simulink model "FullFMS_SIM_V0_1_5_R2025b"  (R2025b)
settings: Solver=FixedStepAuto  StopTime=inf  FixedStep=0.01  MaxStep=0.01  RelTol=1e-2
PreLoadFcn:
  | load("BUS_CONFIG_SIM.mat"); run("Param_SIM_V0_1_5.m")
libraries: opcualib x8
(part 2 of 2)

== stateflow chart FullFMS_SIM_V0_1_5_R2025b/Chart_SIM ==
  settings: updateMethod=DISCRETE  sampleTime=Ts_SIM
  state Conveyor29 [parallel]
    settings: executionOrder=1
    state Idle
      entry: SimSensors_20.SS_29_Cart_Stat=false; SimSensors_20.SS_29_Optic=false; SimSensors_20.SS_29_Cart_Next=false;
    state Arriving
      entry: SimSensors_20.SS_29_Cart_Next=true; SimActuators_20.SA_20_Conveyor=true; SimSensors_20.SS_20_Controler_On=true;
    state AtStop
      entry: SimSensors_20.SS_29_Cart_Next=false; SimSensors_20.SS_29_Count=true; SimSensors_20.SS_29_Cart_Stat=true; SimSensors_20.SS_29_Optic=true;
      PartOnCart=true; CartAt29=true; SimActuators_20.SA_20_Conveyor=false;
    state Delivered
      entry: SimSensors_20.SS_29_Count=false; SimControl_20.SC_29_CartDel=true; CRouteIn54=true; SimASi_50.SR_54_CRoute_In=true;
      during: SimSensors_20.SS_29_Optic = PartOnCart;
    state Leaving
      entry: SimControl_20.SC_29_CartDel=false; CRouteIn54=false; SimASi_50.SR_54_CRoute_In=false; CartAt29=false;
    (default) -> Idle
    Leaving -> Idle : after(t_leave,sec)
    Idle -> Arriving : [nCart < N_PARTS]
    Arriving -> AtStop : after(t_conv,sec)
    AtStop -> Delivered : after(T_CONV_T6,sec)
    Delivered -> Leaving : [SimASi_50.SR_54_CRoute_Out]
  state HD1_Ctrl [parallel]
    settings: executionOrder=2
    state Init
      entry: SimControl_50.SC_52_Profibus=true; SimControl_50.SC_55_PD_Sort=false; SimASi_50.SR_54_CRoute_Out=false;
      SimActuators_50.SA_50_Claw_Down=false; SimActuators_50.SA_50_Close_Claw=false; SimActuators_50.SA_50_Claw_2_Del=false; SimActuators_50.SA_50_Claw_2_Cart=false;
    state Ready
      entry: SimControl_50.SC_55_Initialization=true;
    state N1_StartMove
      entry: SimControl_50.SC_55_PD_Sort=false;
    state N2_LowerClaw
      entry: SimActuators_50.SA_50_Claw_Down=true;
    state N3_CloseClaw
      entry: SimActuators_50.SA_50_Close_Claw=true;
    state N3_Raise
      entry: SimActuators_50.SA_50_Claw_Down=false;
    state N4_Claw2Del
      entry: SimActuators_50.SA_50_Claw_2_Cart=false; SimActuators_50.SA_50_Claw_2_Del=true;
    state N5_LowerClaw2
      entry: SimActuators_50.SA_50_Claw_Down=true;
    state N6_Release
      entry: SimActuators_50.SA_50_Close_Claw=false;
    state N6_Raise
      entry: SimActuators_50.SA_50_Claw_Down=false;
    state N7_PDSort
      entry: SimControl_50.SC_55_PD_Sort=true;
    state N8_Claw2Cart
      entry: SimActuators_50.SA_50_Claw_2_Del=false; SimActuators_50.SA_50_Claw_2_Cart=true; Claw2CartCmd=true;
    state N9_CRouteOut
      entry: SimActuators_50.SA_50_Claw_2_Cart=false; Claw2CartCmd=false; SimASi_50.SR_54_CRoute_Out=true;
      exit: SimASi_50.SR_54_CRoute_Out=false; nCart = nCart + 1;
    (default) -> Init
    Init -> Ready : [SimSensors_50.SS_50_Claw_Cart && SimSensors_50.SS_50_Claw_High && ~SimSensors_50.SS_50_Part_in_Claw]
    N9_CRouteOut -> Ready : after(T_HD1_T1,sec)
    Ready -> N1_StartMove : [CRouteIn54 && CartAt29 && SimSensors_20.SS_29_Optic && ~SimSensors_60.SS_60_SPart]
    N1_StartMove -> N2_LowerClaw : [~SimControl_50.SC_55_PD_Sort && SimSensors_50.SS_50_Claw_Cart && SimSensors_50.SS_50_Claw_High && ~SimSensors_50.SS_50_Part_in_Claw]
    N2_LowerClaw -> N3_CloseClaw : [SimSensors_50.SS_50_Claw_Cart && SimSensors_50.SS_50_Claw_Low]
    N3_CloseClaw -> N3_Raise : [SimSensors_50.SS_50_Part_in_Claw]
    N3_Raise -> N4_Claw2Del : [SimSensors_50.SS_50_Claw_High && SimSensors_50.SS_50_Part_in_Claw && ~SimSensors_50.SS_50_Claw_Del]
    N4_Claw2Del -> N5_LowerClaw2 : [SimSensors_50.SS_50_Claw_Del && SimSensors_50.SS_50_Claw_High && SimSensors_50.SS_50_Part_in_Claw]
    N5_LowerClaw2 -> N6_Release : [SimSensors_50.SS_50_Claw_Del && SimSensors_50.SS_50_Claw_Low]
    N6_Release -> N6_Raise : [~SimSensors_50.SS_50_Part_in_Claw]
    N6_Raise -> N7_PDSort : [SimSensors_50.SS_50_Claw_Del && SimSensors_50.SS_50_Claw_High && ~SimSensors_50.SS_50_Part_in_Claw]
    N7_PDSort -> N8_Claw2Cart
    N8_Claw2Cart -> N9_CRouteOut : [SimSensors_50.SS_50_Claw_Cart]
  state HD1_Plant [parallel]
    settings: executionOrder=3
    state Vertical [parallel]
      settings: executionOrder=1
      state High
        entry: SimSensors_50.SS_50_Claw_High=true; SimSensors_50.SS_50_Claw_Low=false;
      state GoingDown
        entry: SimSensors_50.SS_50_Claw_High=false;
      state Low
        entry: SimSensors_50.SS_50_Claw_Low=true;
      state GoingUp
        entry: SimSensors_50.SS_50_Claw_Low=false;
      (default) -> High
      GoingUp -> High [order 1] : after(t_v_up,sec)
      High -> GoingDown : [SimActuators_50.SA_50_Claw_Down]
      GoingUp -> GoingDown [order 2] : [SimActuators_50.SA_50_Claw_Down]
      GoingDown -> Low [order 1] : after(t_v_down,sec)
      GoingDown -> GoingUp [order 2] : [~SimActuators_50.SA_50_Claw_Down]
      Low -> GoingUp : [~SimActuators_50.SA_50_Claw_Down]
    state Horizontal [parallel]
      settings: executionOrder=2
      state AtCart
        entry: SimSensors_50.SS_50_Claw_Cart=true; SimSensors_50.SS_50_Claw_Del=false;
      state ToDel
        entry: SimSensors_50.SS_50_Claw_Cart=false;
      state AtDel
        entry: SimSensors_50.SS_50_Claw_Del=true;
      state ToCart
        entry: SimSensors_50.SS_50_Claw_Del=false;
      (default) -> AtCart
      ToCart -> AtCart : after(t_h_cart,sec)
      AtCart -> ToDel : [SimActuators_50.SA_50_Claw_2_Del]
      ToDel -> AtDel : after(t_h_del,sec)
      AtDel -> ToCart : [SimActuators_50.SA_50_Claw_2_Cart]
    state Gripper [parallel]
      settings: executionOrder=3
      state Empty
        entry: SimSensors_50.SS_50_Part_in_Claw=false;
      state Gripping
      state Holding
        entry: SimSensors_50.SS_50_Part_in_Claw=true; PartOnCart=false;
      state Releasing
      (default) -> HD1_Plant.Gripper.Empty
      Releasing -> HD1_Plant.Gripper.Empty : after(t_grip,sec){SimSensors_60.SS_60_SPart = SimSensors_60.SS_60_SPart || SimSensors_50.SS_50_Claw_Del;}
      HD1_Plant.Gripper.Empty -> Gripping : [SimActuators_50.SA_50_Close_Claw && SimSensors_50.SS_50_Claw_Low && SimSensors_50.SS_50_Claw_Cart && PartOnCart]
      Gripping -> Holding : after(t_grip,sec)
      Holding -> Releasing : [~SimActuators_50.SA_50_Close_Claw && SimSensors_50.SS_50_Claw_Low]
  state SORT_Ctrl [parallel]
    entry: SimControl_60.SC_62_Profibus=false; SimControl_60.SC_65_Initialization=false; SimControl_60.SC_65_ID_1=false; SimControl_60.SC_65_ID_2=false; SimControl_60.SC_65_Part_Sorted=false;
    SimControl_60.SC_65_RBS_Output = (SORT_MODE == 1); SimControl_60.SC_65_RSB_Output = (SORT_MODE == 2); SimControl_60.SC_65_BRS_Output = (SORT_MODE == 3); SimControl_60.SC_65_BSR_Output = (SORT_MODE == 4); SimControl_60.SC_65_SRB_Output = (SORT_MODE == 5); SimControl_60.SC_65_SBR_Output = (SORT_MODE == 6);
    SimActuators_60.SA_60_Conveyor=false; SimActuators_60.SA_60_P1=false; SimActuators_60.SA_60_P2=false; SimActuators_60.SA_60_Identify=false; SimActuators_60.SA_61_Led_Start=false; SimActuators_60.SA_61_Led_Reset=false; SimActuators_60.SA_61_Led_Extra1=false; SimActuators_60.SA_61_Led_Extra2=false; SimActuators_60.SA_61_Panel_O4=false; SimActuators_60.SA_61_Panel_O5=false; SimActuators_60.SA_61_Panel_O6=false; SimActuators_60.SA_61_Panel_O7=false;
    FBSel = (SORT_MODE == 1 && SimControl_60.SC_65_RBS_Output) || (SORT_MODE == 2 && SimControl_60.SC_65_RSB_Output) || (SORT_MODE == 3 && SimControl_60.SC_65_BRS_Output) || (SORT_MODE == 4 && SimControl_60.SC_65_BSR_Output) || (SORT_MODE == 5 && SimControl_60.SC_65_SRB_Output) || (SORT_MODE == 6 && SimControl_60.SC_65_SBR_Output);
    settings: executionOrder=4
    state FB1_Init [parallel]
      settings: executionOrder=1
      state FB1_N2_Check
        entry: SimControl_60.SC_62_Profibus=true; FB1Init=false; SimControl_60.SC_65_Initialization=false;
      state FB1_N3_ClearPart
        entry: FB1Conv=true; FB1IDPin=true;
      state FB1_N1_InitOk
        entry: FB1Init=true; SimControl_60.SC_65_Initialization=true;
      (default) -> SORT_Ctrl.FB1_Init.FB1_N2_Check
      FB1_N3_ClearPart -> SORT_Ctrl.FB1_Init.FB1_N2_Check : [FB1Conv && SimSensors_60.SS_60_Part_Pass]{FB1Conv=false; FB1IDPin=false;}
      FB1_N1_InitOk -> SORT_Ctrl.FB1_Init.FB1_N2_Check : [SimSensors_60.SS_61_Reset]{FB1Conv=false; FB1IDPin=false; TrigConv=false; Lever1=false; Lever2=false; PinSort=false; PartDel=false;}
      SORT_Ctrl.FB1_Init.FB1_N2_Check -> FB1_N1_InitOk [order 1] : [SimControl_60.SC_62_Profibus && ~FB1Conv && ~SimSensors_60.SS_60_SPart && ~SimSensors_60.SS_60_SInd && ~SimSensors_60.SS_60_SPhoto && ~SimSensors_60.SS_60_Part_Pass]
      SORT_Ctrl.FB1_Init.FB1_N2_Check -> FB1_N3_ClearPart [order 2] : [SimSensors_60.SS_60_SPart || SimSensors_60.SS_60_SInd || SimSensors_60.SS_60_SPhoto]
    state FB4_9_Sort [parallel]
      settings: executionOrder=2
      state OB1_N4_9_Select
      state N1_StartConv
        entry: TrigConv=true; SimControl_60.SC_65_ID_1=false; SimControl_60.SC_65_ID_2=false;
      state N2_Identify
        en, du: if SimSensors_60.SS_60_SInd, SimControl_60.SC_65_ID_1=false; SimControl_60.SC_65_ID_2=true;
        elseif SimSensors_60.SS_60_SPhoto, SimControl_60.SC_65_ID_1=true; SimControl_60.SC_65_ID_2=true;
        else, SimControl_60.SC_65_ID_1=true; SimControl_60.SC_65_ID_2=false; end
      state N3_SelectLever
        entry: cID = 0;
        if SimControl_60.SC_65_ID_1 && SimControl_60.SC_65_ID_2, cID = 1; elseif SimControl_60.SC_65_ID_1, cID = 2; elseif SimControl_60.SC_65_ID_2, cID = 3; end
        Lever1 = (cID == SORT_MAP(SORT_MODE,1)); Lever2 = (cID == SORT_MAP(SORT_MODE,2)); PassStr = (cID == SORT_MAP(SORT_MODE,3));
        during: if (Lever1 && SimSensors_60.SS_60_SL1_Fwd) || (Lever2 && SimSensors_60.SS_60_SL2_Fwd) || (PassStr && SimSensors_60.SS_60_SL1_Bck && SimSensors_60.SS_60_SL2_Bck), PinSort = true; end
      state N4_PartDel
        entry: PartDel=true; Lever1=false;
        if SORT_MODE ~= 3, Lever2=false; end
      state N5_ResetNext
        entry: TrigConv=false; PinSort=false; PartDel=false; Lever1=false; Lever2=false; PassStr=false;
      (default) -> OB1_N4_9_Select
      N5_ResetNext -> OB1_N4_9_Select
      OB1_N4_9_Select -> N1_StartConv : [FB1Init && FBSel && SimControl_50.SC_55_PD_Sort && SimSensors_50.SS_50_Claw_Del]
      N1_StartConv -> N2_Identify
      N2_Identify -> N3_SelectLever : after(T_SORT_ID - Ts_SIM,sec)
      N3_SelectLever -> N4_PartDel : [SimSensors_60.SS_60_Part_Pass]
      N4_PartDel -> N5_ResetNext
    state OB1_N10_11 [parallel]
      settings: executionOrder=3
      state N10_Wait
        entry: SimControl_60.SC_65_Part_Sorted=false;
      state N10_PartPass
      state N11_PartSorted
        entry: SimControl_60.SC_65_Part_Sorted=true;
      (default) -> N10_Wait
      N11_PartSorted -> N10_Wait : after(T_SORT_T7,sec)
      N10_Wait -> N10_PartPass : [SimSensors_60.SS_60_Part_Pass]
      N10_PartPass -> N11_PartSorted : [~SimSensors_60.SS_60_Part_Pass]
    state FB3_Actuators [parallel]
      settings: executionOrder=4
      state FB3_Map
        during: ConvOn60 = SimSensors_60.SS_61_Key_Pos && (TrigConv || FB1Conv); SimActuators_60.SA_60_Conveyor = ConvOn60;
        SimActuators_60.SA_60_P1 = SimSensors_60.SS_61_Key_Pos && Lever1; SimActuators_60.SA_60_P2 = SimSensors_60.SS_61_Key_Pos && Lever2;
        SimActuators_60.SA_60_Identify = SimSensors_60.SS_61_Key_Pos && (PinSort || FB1IDPin);
        SimActuators_60.SA_61_Led_Start = SimSensors_60.SS_61_Key_Pos && FB1Init; SimActuators_60.SA_61_Led_Reset = SimSensors_60.SS_61_Key_Pos && SimSensors_60.SS_61_Reset;
        SimActuators_60.SA_61_Led_Extra1 = SimControl_60.SC_65_Part_Sorted; SimActuators_60.SA_61_Led_Extra2 = false;
        SimActuators_60.SA_61_Panel_O4 = false; SimActuators_60.SA_61_Panel_O5 = false; SimActuators_60.SA_61_Panel_O6 = false; SimActuators_60.SA_61_Panel_O7 = false;
      (default) -> SORT_Ctrl.FB3_Actuators.FB3_Map
  state SORT_Plant [parallel]
    entry: SimSensors_60.SS_60_SPart=false; SimSensors_60.SS_60_SInd=false; SimSensors_60.SS_60_SPhoto=false; SimSensors_60.SS_60_Part_Pass=false;
    SimSensors_60.SS_60_SL1_Bck=true; SimSensors_60.SS_60_SL1_Fwd=false; SimSensors_60.SS_60_SL2_Bck=true; SimSensors_60.SS_60_SL2_Fwd=false;
    SimSensors_60.SS_61_Key_Pos=true; SimSensors_60.SS_61_Start=false; SimSensors_60.SS_61_Stop=false; SimSensors_60.SS_61_Reset=false;
    SimSensors_60.SS_61_Panel_I4=false; SimSensors_60.SS_61_Panel_I5=false; SimSensors_60.SS_61_Panel_I6=false; SimSensors_60.SS_61_Panel_I7=false;
    settings: executionOrder=5
    state Part [parallel]
      settings: executionOrder=1
      state Empty
        entry: SimSensors_60.SS_60_Part_Pass=false;
      state AtEntry
        entry: sortColor = PART_COLORS(min(nSortIn+1, numel(PART_COLORS))); nSortIn = nSortIn + 1;
      state ToStopper
        entry: xSort = 0;
        during: if ConvOn60, xSort = xSort + Ts_SIM; end
        SimSensors_60.SS_60_SPart = xSort < t_s_spart_off;
        if xSort >= t_s_photo, SimSensors_60.SS_60_SPhoto = (sortColor ~= 2); end
        if xSort >= t_s_ind, SimSensors_60.SS_60_SInd = (sortColor == 3); end
      state AtStopper
      state Released
        entry: xSort = 0;
        if SimSensors_60.SS_60_SL1_Fwd, sortExit = 1; elseif SimSensors_60.SS_60_SL2_Fwd, sortExit = 2; else, sortExit = 3; end
        during: if ConvOn60, xSort = xSort + Ts_SIM; end
        if xSort >= t_s_ind_off, SimSensors_60.SS_60_SInd = false; end
        if xSort >= t_s_photo_off, SimSensors_60.SS_60_SPhoto = false; end
      state PartPass
        entry: SimSensors_60.SS_60_Part_Pass = true; SimSensors_60.SS_60_SInd = false; SimSensors_60.SS_60_SPhoto = false; nDone = nDone + 1;
      (default) -> SORT_Plant.Part.Empty
      PartPass -> SORT_Plant.Part.Empty : after(t_s_pp,sec)
      SORT_Plant.Part.Empty -> AtEntry : [SimSensors_60.SS_60_SPart]
      AtEntry -> ToStopper : [SimActuators_60.SA_60_Conveyor]
      ToStopper -> AtStopper : [xSort >= t_s_ind]
      AtStopper -> Released : [SimActuators_60.SA_60_Identify && SimActuators_60.SA_60_Conveyor]
      Released -> PartPass : [(sortExit == 1 && xSort >= t_s_pass1) || (sortExit == 2 && xSort >= t_s_pass2) || (sortExit == 3 && xSort >= t_s_pass3)]
    state Lever1 [parallel]
      settings: executionOrder=2
      state SL1_Bck
        entry: SimSensors_60.SS_60_SL1_Bck=true; SimSensors_60.SS_60_SL1_Fwd=false;
      state SL1_ToFwd
        entry: SimSensors_60.SS_60_SL1_Bck=false;
      state SL1_Fwd
        entry: SimSensors_60.SS_60_SL1_Fwd=true;
      state SL1_ToBck
        entry: SimSensors_60.SS_60_SL1_Fwd=false;
      (default) -> SL1_Bck
      SL1_ToBck -> SL1_Bck [order 1] : after(t_sl1_bck,sec)
      SL1_Bck -> SL1_ToFwd : [SimActuators_60.SA_60_P1]
      SL1_ToBck -> SL1_ToFwd [order 2] : [SimActuators_60.SA_60_P1]
      SL1_ToFwd -> SL1_Fwd [order 1] : after(t_sl1_fwd,sec)
      SL1_ToFwd -> SL1_ToBck [order 2] : [~SimActuators_60.SA_60_P1]
      SL1_Fwd -> SL1_ToBck : [~SimActuators_60.SA_60_P1]
    state Lever2 [parallel]
      settings: executionOrder=3
      state SL2_Bck
        entry: SimSensors_60.SS_60_SL2_Bck=true; SimSensors_60.SS_60_SL2_Fwd=false;
      state SL2_ToFwd
        entry: SimSensors_60.SS_60_SL2_Bck=false;
      state SL2_Fwd
        entry: SimSensors_60.SS_60_SL2_Fwd=true;
      state SL2_ToBck
        entry: SimSensors_60.SS_60_SL2_Fwd=false;
      (default) -> SL2_Bck
      SL2_ToBck -> SL2_Bck [order 1] : after(t_sl2_bck,sec)
      SL2_Bck -> SL2_ToFwd : [SimActuators_60.SA_60_P2]
      SL2_ToBck -> SL2_ToFwd [order 2] : [SimActuators_60.SA_60_P2]
      SL2_ToFwd -> SL2_Fwd [order 1] : after(t_sl2_fwd,sec)
      SL2_ToFwd -> SL2_ToBck [order 2] : [~SimActuators_60.SA_60_P2]
      SL2_Fwd -> SL2_ToBck : [~SimActuators_60.SA_60_P2]
  state TEST_Ctrl [parallel]
    entry: SimControl_70.SC_72_Profibus=false; SimControl_70.SC_75_Initialization=false; SimControl_70.SC_75_RQ_Delivery1=false; SimControl_70.SC_75_ID_Delivery1=false; SimControl_70.SC_75_RQ_Delivery2=false; SimControl_70.SC_75_ID_Delivery2=false; SimControl_70.SC_75_Part_Del=false; SimControl_70.SC_75_RQ_Part_Del=false; SimControl_70.SC_75_RQ_Wrong=false;
    SimControl_70.SC_75_Identified = (TEST_MODE == 1); SimControl_70.SC_75_Requested = (TEST_MODE == 2); SimControl_70.SC_75_Identified80 = (TEST_MODE == 1); SimControl_70.SC_75_Requested80 = (TEST_MODE == 2);
    SimActuators_70.SA_70_Elev_Down=false; SimActuators_70.SA_70_Elev_Up=false; SimActuators_70.SA_70_Eject_Part=false; SimActuators_70.SA_70_Air_On=false; SimActuators_70.SA_71_Led_Start=false; SimActuators_70.SA_71_Led_Reset=false; SimActuators_70.SA_71_Led_Extra1=false; SimActuators_70.SA_71_Led_Extra2=false; SimActuators_70.SA_71_Panel_O4=false; SimActuators_70.SA_71_Panel_O5=false; SimActuators_70.SA_71_Panel_O6=false; SimActuators_70.SA_71_Panel_O7=false;
    SimASi_70.SR_73_TestCartID=0; SimASi_70.SR_74_Request=false; SimASi_70.SR_74_No_Cart=true; SimASi_70.SR_74_Cart_Full=false; SimASi_70.SR_74_CRoute_Out=false; SimASi_70.SR_74_CRoute_In=false;
    settings: executionOrder=6
    state FB1_Init70 [parallel]
      settings: executionOrder=1
      state FB1_N2_N3_Check
        entry: SimControl_70.SC_72_Profibus=true; FB1Init70=false; SimControl_70.SC_75_Initialization=false;
        during: FB1ElevDown70 = ~ElevLow70;
      state FB1_N3_PistonPulse
        entry: FB1PistAdv70=true;
      state FB1_N1_N4_InitOk
        entry: FB1Init70=true; SimControl_70.SC_75_Initialization=true; FB1ElevDown70=false; FB1PistAdv70=false;
      (default) -> FB1_N2_N3_Check
      FB1_N3_PistonPulse -> FB1_N2_N3_Check : after(T_TEST_T1,sec){FB1PistAdv70=false;}
      FB1_N1_N4_InitOk -> FB1_N2_N3_Check : [SimSensors_70.SS_71_Reset]{IdenDel=false; IdenProc=false; EjectProc=false; ReturnElev=false; ReqDel=false; IdenColor=false; PartOk=false; EjectOk=false; PartDiff=false; EjectBad=false;}
      FB1_N2_N3_Check -> FB1_N1_N4_InitOk [order 1] : [~PartIn70 && ElevLow70 && PistBck70 && DistInit85]
      FB1_N2_N3_Check -> FB1_N3_PistonPulse [order 2] : [ElevLow70 && PartIn70]
    state FB4_Identified [parallel]
      settings: executionOrder=2
      state OB1_N4_Off
      state FB4_Wait
      state N1_StartID
        entry: IdenDel=true; idA70=false; idB70=false; PartDel70=false; RQPartDel70=false;
      state N2_N3_Raise
        en, du: if PartIn70 && ElevLow70 && SInd70, idB70 = true; end
        FB4ElevUp = PartIn70 && PistBck70 && ArmMag80;
      state N4_Identify
        entry: IdenProc=true; FB4ElevUp=true;
        en, du: if ~idB70, idA70 = true; if Height70, idB70 = true; end; end
      state N5_EjectWaitCart
        entry: IdenProc=false; EjectProc=true; FB4ElevUp=true;
      state N5_EjectPush
        entry: FB4PistFwd=true; FB4Air=true;
      state N5_EjectEnd
        entry: FB4PistFwd=false; FB4Air=false;
        en, du: FB4CartFull = CartStat24 && Optic24 && ~PistBck24;
      state N6_ReturnElev
        entry: EjectProc=false; ReturnElev=true; FB4ElevUp=false; FB4CartFull=false; FB4ElevDown=ArmMag80;
      state N6_PartDel
        entry: FB4ElevDown=false; PartDel70=true; ReturnElev=false;
      (default) -> OB1_N4_Off
      OB1_N4_Off -> TEST_Ctrl.FB4_Identified.FB4_Wait : [FB1Init70 && SimControl_70.SC_75_Identified]
      N6_PartDel -> TEST_Ctrl.FB4_Identified.FB4_Wait
      TEST_Ctrl.FB4_Identified.FB4_Wait -> N1_StartID : [PartIn70]
      N1_StartID -> TEST_Ctrl.FB4_Identified.N2_N3_Raise
      TEST_Ctrl.FB4_Identified.N2_N3_Raise -> N4_Identify : [ElevHigh70 && FB4ElevUp]
      N4_Identify -> N5_EjectWaitCart : after(T_TEST_T2,sec)
      N5_EjectWaitCart -> N5_EjectPush : [~PistBck24 && CartStat24 && ~Optic24]
      N5_EjectPush -> N5_EjectEnd [order 1] : [Optic24]
      N5_EjectPush -> N5_EjectEnd [order 2] : after(T_TEST_T3,sec)
      N5_EjectEnd -> N6_ReturnElev : [PistBck70 && ~PartIn70 && Optic24]
      N6_ReturnElev -> N6_PartDel : [ElevLow70]
    state FB5_Requested [parallel]
      settings: executionOrder=3
      state OB1_N5_Off
      state FB5_Wait
      state N1_StartReq
        entry: ReqDel=true; PartDiff=false; idA70=false; idB70=false; PartDel70=false; RQPartDel70=false; RQWrong70=false;
      state N2_N3_Raise
        en, du: if PartIn70 && ElevLow70 && SInd70, idB70 = true; end
        FB5ElevUp = PartIn70 && PistBck70 && ArmMag80 && ~PartDiff;
      state N4_ColorWindow
        entry: IdenColor=true; FB5ElevUp=true;
        en, du: if ~idB70, idA70 = true; if Height70, idB70 = true; end; end
      state N4_ColorHold
      state N5_Compare
        entry: IdenColor=false; FB5ElevUp=false;
        if (idA70 == RQ1_70) && (idB70 == RQ2_70), PartOk=true; EjectOk=true;
        else, PartDiff=true; EjectBad=true; end
      state N6_EjectWaitCart
      state N6_EjectPush
        entry: FB5PistFwd1=true; FB5Air=true;
      state N6_EjectEnd
        entry: FB5PistFwd1=false; FB5Air=false;
        en, du: FB5CartFull = CartStat24 && Optic24 && ~PistBck24;
      state N7_ReturnElev
        entry: EjectOk=false; ReturnElev=true; FB5CartFull=false; FB5ElevDown1=ArmMag80;
      state N7_RQPartDel
        entry: FB5ElevDown1=false; RQPartDel70=true; ReturnElev=false; PartOk=false;
      state N10_ResetReq
        entry: ReqDel=false;
      state N8_DownBad
        entry: FB5ElevDown2=ArmMag80;
      state N8_EjectBad
        entry: FB5ElevDown2=false; FB5PistFwd2=true;
      state N8_WaitBack
        entry: FB5PistFwd2=false;
      state N9_RQWrong
        entry: EjectBad=false; RQWrong70=true;
      (default) -> TEST_Ctrl.FB5_Requested.OB1_N5_Off
      TEST_Ctrl.FB5_Requested.OB1_N5_Off -> TEST_Ctrl.FB5_Requested.FB5_Wait : [FB1Init70 && SimControl_70.SC_75_Requested]
      N10_ResetReq -> TEST_Ctrl.FB5_Requested.FB5_Wait
      N9_RQWrong -> TEST_Ctrl.FB5_Requested.FB5_Wait
      TEST_Ctrl.FB5_Requested.FB5_Wait -> N1_StartReq : [PartIn70]
      N1_StartReq -> TEST_Ctrl.FB5_Requested.N2_N3_Raise
      TEST_Ctrl.FB5_Requested.N2_N3_Raise -> N4_ColorWindow : [ElevHigh70 && FB5ElevUp]
      N4_ColorWindow -> N4_ColorHold : after(T_TEST_T8,sec)
      N4_ColorHold -> N5_Compare : after(T_TEST_T2 - T_TEST_T8,sec)
      N5_Compare -> N6_EjectWaitCart [order 1] : [PartOk]
      N5_Compare -> N8_DownBad [order 2] : [PartDiff]
      N6_EjectWaitCart -> N6_EjectPush : [~PistBck24 && CartStat24 && ~Optic24]
      N6_EjectPush -> N6_EjectEnd [order 1] : [Optic24]
      N6_EjectPush -> N6_EjectEnd [order 2] : after(T_TEST_T5,sec)
      N6_EjectEnd -> N7_ReturnElev : [PistBck70 && ~PartIn70 && Optic24]
      N7_ReturnElev -> N7_RQPartDel : [ElevLow70]
      N7_RQPartDel -> N10_ResetReq
      N8_DownBad -> N8_EjectBad : [ElevLow70]
      N8_EjectBad -> N8_WaitBack : after(T_TEST_T6,sec)
      N8_WaitBack -> N9_RQWrong : [PistBck70 && ~PartIn70]
    state OB1_N6_Routing [parallel]
      settings: executionOrder=4
      state OB1_N6_Wait
      state OB1_N6_T7_CRouteOut
        entry: SimASi_70.SR_74_CRoute_Out=true; RouteOut74=true;
      state OB1_N6_Hold
        entry: SimASi_70.SR_74_CRoute_Out=false; RouteOut74=false;
      (default) -> OB1_N6_Wait
      OB1_N6_Hold -> OB1_N6_Wait : [~PartDel70 && ~RQPartDel70]
      OB1_N6_Wait -> OB1_N6_T7_CRouteOut : [PartDel70 || RQPartDel70]
      OB1_N6_T7_CRouteOut -> OB1_N6_Hold : after(T_TEST_T7,sec)
    state FB3_OB1_Map [parallel]
      settings: executionOrder=5
      state FB3_Map
        during: ElevUp70 = KeyPos71 && (FB4ElevUp || FB5ElevUp);
        ElevDown70 = KeyPos71 && (FB1ElevDown70 || FB4ElevDown || FB5ElevDown1 || FB5ElevDown2);
        Eject70 = KeyPos71 && (FB1PistAdv70 || FB4PistFwd || FB5PistFwd1 || FB5PistFwd2);
        Air70 = KeyPos71 && (FB4Air || FB5Air);
        SimActuators_70.SA_70_Elev_Up = ElevUp70; SimActuators_70.SA_70_Elev_Down = ElevDown70; SimActuators_70.SA_70_Eject_Part = Eject70; SimActuators_70.SA_70_Air_On = Air70;
        NoCart74 = ~CartStat24; CartFull74 = (FB4CartFull && TEST_MODE == 1) || (FB5CartFull && TEST_MODE == 2) || (CartStat24 && Optic24);
        SimASi_70.SR_74_No_Cart = NoCart74; SimASi_70.SR_74_Cart_Full = CartFull74; CRouteIn80 = CRouteIn74;
        SimActuators_70.SA_71_Led_Start = KeyPos71 && FB1Init70; SimActuators_70.SA_71_Led_Extra1 = NoCart74; SimActuators_70.SA_71_Led_Extra2 = CartFull74;
        SimControl_70.SC_75_ID_Delivery1 = idA70; SimControl_70.SC_75_ID_Delivery2 = idB70; SimControl_70.SC_75_Part_Del = PartDel70;
        SimControl_70.SC_75_RQ_Part_Del = RQPartDel70; SimControl_70.SC_75_RQ_Wrong = RQWrong70;
      (default) -> TEST_Ctrl.FB3_OB1_Map.FB3_Map
  state TEST_Plant [parallel]
    entry: KeyPos71=true; ElevLow70=true; PistBck70=true;
    SimSensors_70.SS_71_Key_Pos=true; SimSensors_70.SS_71_Start=false; SimSensors_70.SS_71_Stop=false; SimSensors_70.SS_71_Reset=false;
    SimSensors_70.SS_71_Panel_I4=false; SimSensors_70.SS_71_Panel_I5=false; SimSensors_70.SS_71_Panel_I6=false; SimSensors_70.SS_71_Panel_I7=false;
    settings: executionOrder=7
    state Elevator [parallel]
      settings: executionOrder=1
      state Elev_Low
        entry: ElevLow70=true; ElevHigh70=false; SInd70 = PartIn70 && testColor == 3; SStation70=false;
      state Elev_GoingUp
        entry: tElev = 0;
        during: tElev = tElev + Ts_SIM; ElevLow70 = tElev < t_t_up_lowoff;
        SInd70 = (PartIn70 && testColor == 3 && tElev < t_t_metal_off) || (tElev >= t_t_up_ind && tElev < t_t_up_ind + 0.15);
        SStation70 = tElev >= t_t_up_sst && tElev < t_t_up_sst + 0.22;
        Height70 = PartIn70 && testColor ~= 2 && tElev >= t_t_up - t_t_height_pre;
      state Elev_High
        entry: ElevHigh70=true; ElevLow70=false; SInd70=false; SStation70=false; Height70 = PartIn70 && testColor ~= 2;
      state Elev_GoingDown
        entry: tElev = 0; Height70=false;
        during: tElev = tElev + Ts_SIM; ElevHigh70 = tElev < t_t_down_highoff;
        SStation70 = tElev >= t_t_down_sst && tElev < t_t_down_sst + 0.27;
        SInd70 = (tElev >= t_t_down_ind && tElev < t_t_down_ind + 0.18) || (PartIn70 && testColor == 3 && tElev >= t_t_down - 0.3);
      (default) -> Elev_Low
      Elev_GoingDown -> Elev_Low [order 1] : [tElev >= t_t_down]
      Elev_Low -> Elev_GoingUp : [ElevUp70 && ~ElevDown70]
      Elev_GoingDown -> Elev_GoingUp [order 2] : [ElevUp70 && ~ElevDown70]
      Elev_GoingUp -> Elev_High [order 1] : [tElev >= t_t_up]
      Elev_GoingUp -> Elev_GoingDown [order 2] : [ElevDown70]
      Elev_High -> Elev_GoingDown : [ElevDown70]
    state SlideToCart [parallel]
      settings: executionOrder=3
      state Slide_Empty
      state Slide_Moving
        entry: PartToCart=false;
      state Slide_OnCart
        entry: if CartStat24, SimSensors_20.SS_24_Optic=true; Optic24=true; CartHasPart=true; end
      (default) -> Slide_Empty
      Slide_OnCart -> Slide_Empty
      Slide_Empty -> Slide_Moving : [PartToCart]
      Slide_Moving -> Slide_OnCart : after(t_t_ej_cart - t_t_ej_spart,sec)
    state Sensors_Out [parallel]
      settings: executionOrder=4
      state S70_Map
        en, du: SimSensors_70.SS_70_SPart = PartIn70; SimSensors_70.SS_70_Elev_Low = ElevLow70; SimSensors_70.SS_70_Elev_High = ElevHigh70;
        SimSensors_70.SS_70_SInductive = SInd70; SimSensors_70.SS_70_SPart_Height = Height70; SimSensors_70.SS_70_Pist_Bck = PistBck70;
        SimSensors_70.SS_70_SStation = SStation70;
      (default) -> S70_Map
    state Piston [parallel]
      settings: executionOrder=2
      state Pist_Back
        entry: PistBck70=true;
      state Pist_Fwd
        entry: tPist = 0;
        during: tPist = tPist + Ts_SIM; PistBck70 = tPist < t_t_pist_fwd;
        if PartIn70 && tPist >= t_t_ej_spart
        PartIn70 = false; Height70 = false; SInd70 = false;
        if ElevHigh70, PartToCart = true; else, nReject = nReject + 1; end
        end
      state Pist_Return
        entry: PistBck70=false;
      (default) -> Pist_Back
      Pist_Return -> Pist_Back : after(t_t_pist_back,sec)
      Pist_Back -> Pist_Fwd : [Eject70]
      Pist_Fwd -> Pist_Return : [~Eject70]
  state Conveyor24 [parallel]
    settings: executionOrder=8
    state C24_Idle
      entry: SimSensors_20.SS_24_Cart_Stat=false; SimSensors_20.SS_24_Cart_Next=false; SimSensors_20.SS_24_Count=false; SimSensors_20.SS_24_Optic=false; SimSensors_20.SS_24_Pist_Bck=true;
      SimControl_20.SC_24_Request=false; SimControl_20.SC_24_CartDel=false; SimControl_20.SC_24_CRoute_In=false; SimControl_20.SC_24_CRoute_Out=false;
      CartStat24=false; Optic24=false; PistBck24=true; CartHasPart=false; CRouteIn74=false;
    state C24_Request
      entry: SimControl_20.SC_24_Request=true;
    state C24_Moving
      entry: SimControl_20.SC_24_Request=false;
    state C24_Count
      entry: SimSensors_20.SS_24_Count=true; SimSensors_20.SS_24_Cart_Next=true;
    state C24_N6_AtStop
      entry: SimSensors_20.SS_24_Count=false; SimSensors_20.SS_24_Cart_Next=false; SimSensors_20.SS_24_Cart_Stat=true; SimSensors_20.SS_24_Pist_Bck=false;
      CartStat24=true; PistBck24=false; SimControl_20.SC_24_CartDel=true; SimASi_70.SR_73_TestCartID = nTest + 1;
      RQ1_70 = RQ_DELIVERY(min(nTest + 1, size(RQ_DELIVERY,1)), 1) == 1; RQ2_70 = RQ_DELIVERY(min(nTest + 1, size(RQ_DELIVERY,1)), 2) == 1;
      SimControl_70.SC_75_RQ_Delivery1 = RQ1_70; SimControl_70.SC_75_RQ_Delivery2 = RQ2_70;
    state C24_CRouteIn
      entry: SimASi_70.SR_74_CRoute_In=true; SimControl_20.SC_24_CRoute_In=true; CRouteIn74=true;
    state C24_Docked
      entry: SimASi_70.SR_74_CRoute_In=false; SimControl_20.SC_24_CRoute_In=false; CRouteIn74=false;
    state C24_N7_CartDelOff
      entry: SimControl_20.SC_24_CartDel=false;
    state C24_Release
      entry: SimControl_20.SC_24_CRoute_Out=true;
    state C24_PinBack
      entry: SimSensors_20.SS_24_Pist_Bck=true; PistBck24=true;
    state C24_Leaving
      entry: SimSensors_20.SS_24_Optic=false; Optic24=false;
    state C24_Gone
      entry: SimSensors_20.SS_24_Cart_Stat=false; CartStat24=false; SimControl_20.SC_24_CRoute_Out=false;
      if CartHasPart, nTest = nTest + 1; end
    (default) -> C24_Idle
    C24_Gone -> C24_Idle
    C24_Idle -> C24_Request : [nTest < N_PARTS && FB1Init70]
    C24_Request -> C24_Moving : after(t_24_req,sec)
    C24_Moving -> C24_Count : after(t_24_arrive - t_24_req - t_24_count,sec)
    C24_Count -> C24_N6_AtStop : after(t_24_count,sec)
    C24_N6_AtStop -> C24_CRouteIn : after(t_24_croute_in0,sec)
    C24_CRouteIn -> C24_Docked : after(t_24_croute_in,sec)
    C24_Docked -> C24_N7_CartDelOff : after(T_CONV24_T1 - t_24_croute_in0 - t_24_croute_in,sec)
    C24_N7_CartDelOff -> C24_Release : [RouteOut74]
    C24_Release -> C24_PinBack : after(t_24_pist_bck,sec)
    C24_PinBack -> C24_Leaving : after(t_24_optic_off - t_24_pist_bck,sec)
    C24_Leaving -> C24_Gone : after(t_24_leave - t_24_optic_off,sec)
  state DIST_Ctrl [parallel]
    entry: SimControl_80.SC_82_Profibus=false; SimControl_80.SC_85_Initialization=false; SimControl_80.SC_85_Start=false; SimControl_80.SC_85_Part_Del=false;
    SimControl_80.SC_85_Single = (DIST_MODE == 1); SimControl_80.SC_85_Continuous = (DIST_MODE == 2); SimControl_80.SC_85_Counted = (DIST_MODE == 3);
    SimControl_80.SC_85_Part_Mag=false; SimControl_80.SC_83_RQ_Parts = RQ_PARTS; SimControl_80.SC_86_Mag_Parts = 0; SimControl_80.SC_87_RQ_MParts = 0;
    SimActuators_80.SA_80_Pist_Adv=false; SimActuators_80.SA_80_Suction_On=false; SimActuators_80.SA_80_Suction_Off=false; SimActuators_80.SA_80_Arm_2_Del=false; SimActuators_80.SA_80_Arm_2_Mag=false; SimActuators_80.SA_81_Led_Start=false; SimActuators_80.SA_81_Led_Reset=false; SimActuators_80.SA_81_Led_Extra1=false; SimActuators_80.SA_81_Led_Extra2=false; SimActuators_80.SA_81_Panel_O4=false; SimActuators_80.SA_81_Panel_O5=false; SimActuators_80.SA_81_Panel_O6=false; SimActuators_80.SA_81_Panel_O7=false;
    settings: executionOrder=9
    state FB1_Init80 [parallel]
      settings: executionOrder=1
      state FB1_N2_Check
        entry: SimControl_80.SC_82_Profibus=true; DistInit85=false; SimControl_80.SC_85_Initialization=false;
      state FB1_N3_N4_EmptyMag
        entry: DistInit85=false;
      state FB1_N5_ArmToMag
        en, du: FB1A2M2_80 = ~ArmMag80;
      state FB1_N1_N5_InitOk
        entry: FB1A2M2_80=false; DistInit85=true; SimControl_80.SC_85_Initialization=true;
      (default) -> DIST_Ctrl.FB1_Init80.FB1_N2_Check
      FB1_N1_N5_InitOk -> DIST_Ctrl.FB1_Init80.FB1_N2_Check : [SimSensors_80.SS_81_Reset]
      DIST_Ctrl.FB1_Init80.FB1_N2_Check -> FB1_N5_ArmToMag [order 1] : [MagEmpty80 || MagFull80]{FB1MagEmpty80 = MagEmpty80; FB1MagFull80 = MagFull80;}
      DIST_Ctrl.FB1_Init80.FB1_N2_Check -> FB1_N3_N4_EmptyMag [order 2] : [~MagEmpty80 && ~MagFull80]
      FB1_N5_ArmToMag -> FB1_N1_N5_InitOk : [ArmMag80 && SimControl_80.SC_82_Profibus]
    state OB1_N4_N6_Counter [parallel]
      settings: executionOrder=2
      state OB1_N4_C1
        en, du: if MagFull80 && ~prevMagFull80, cnt80 = cnt80 + 1; end
        if PistFwd80 && ~prevPistFwd80, cnt80 = max(cnt80 - 1, 0); end
        if MagFull80, tMagFull = tMagFull + Ts_SIM; else, tMagFull = 0; end
        if tMagFull >= T_DIST_T1 && tMagFull < T_DIST_T1 + Ts_SIM, cnt80 = 9; end
        if PistBck80 && MagEmpty80, tMagEmpty = tMagEmpty + Ts_SIM; else, tMagEmpty = 0; end
        if tMagEmpty >= T_DIST_T2, cnt80 = 0; end
        prevMagFull80 = MagFull80; prevPistFwd80 = PistFwd80; PartinMag80 = cnt80 > 0;
        SimControl_80.SC_85_Part_Mag = PartinMag80; SimControl_80.SC_86_Mag_Parts = cnt80; SimControl_80.SC_87_RQ_MParts = cnt87;
      (default) -> OB1_N4_C1
    state FB4_Single [parallel]
      settings: executionOrder=4
      state OB1_N7_Off
      state FB4_Wait
      state FB4_N1_SingleOn
        entry: D4On=true;
      state D4_A2D_1
        en, du: D4A2D1 = ~ArmDel80 && ElevLow70 && ~PartIn70;
      state D4_PistFwd
        entry: D4A2D1=false; D4PistFwd=true;
      state D4_Transport
        entry: D4Transport=true; D4PistFwd=false;
      state D4_A2M_1
        en, du: D4A2M1 = ~ArmMag80;
      state D4_SuctOn
        entry: D4A2M1=false; D4SuctOn=true;
      state D4_PartStuck
        entry: D4PartStuckM=true;
      state D4_A2D_2
        en, du: D4A2D2 = ~ArmDel80 && ElevLow70 && ~PartIn70;
      state D4_SuctOff
        entry: D4A2D2=false; D4SuctOn=false;
        en, du: D4SuctOff = PartStuck80;
      state D4_PartDel
        entry: D4SuctOff=false; D4PartDel=true; D4Transport=false; D4PartStuckM=false;
      state D4_A2M_2
        en, du: D4A2M2 = ~ArmMag80;
      state D4_Reset
        entry: D4A2M2=false; D4On=false; D4PartDel=false;
      (default) -> DIST_Ctrl.FB4_Single.OB1_N7_Off
      DIST_Ctrl.FB4_Single.OB1_N7_Off -> DIST_Ctrl.FB4_Single.FB4_Wait : [DistInit85 && SimControl_80.SC_85_Single]
      D4_Reset -> DIST_Ctrl.FB4_Single.FB4_Wait
      DIST_Ctrl.FB4_Single.FB4_Wait -> FB4_N1_SingleOn : [(SimSensors_80.SS_81_Start || SimControl_80.SC_85_Start || RQWrong70 || (CRouteIn80 && KeyPos81)) && ElevLow70 && ~PartIn70 && PartinMag80]
      FB4_N1_SingleOn -> D4_A2D_1
      D4_A2D_1 -> D4_PistFwd : [ArmDel80 && PistBck80]
      D4_PistFwd -> D4_Transport : [PistFwd80]
      D4_Transport -> D4_A2M_1
      D4_A2M_1 -> D4_SuctOn : [ArmMag80]
      D4_SuctOn -> D4_PartStuck : [PartStuck80]
      D4_PartStuck -> D4_A2D_2
      D4_A2D_2 -> D4_SuctOff : [ArmDel80]
      D4_SuctOff -> D4_PartDel : [~PartStuck80]
      D4_PartDel -> D4_A2M_2
      D4_A2M_2 -> D4_Reset : [ArmMag80]
    state FB5_Continuous [parallel]
      settings: executionOrder=5
      state OB1_N8_Off
      state FB5_Wait
      state FB5_N1_AutoOn
        entry: D5On=true;
      state D5_A2D_1
        en, du: D5A2D1 = ~ArmDel80 && ElevLow70 && ~PartIn70;
      state D5_PistFwd
        entry: D5A2D1=false; D5PistFwd=true;
      state D5_Transport
        entry: D5Transport=true; D5PistFwd=false;
      state D5_A2M_1
        en, du: D5A2M1 = ~ArmMag80;
      state D5_SuctOn
        entry: D5A2M1=false; D5SuctOn=true;
      state D5_PartStuck
        entry: D5PartStuckM=true;
      state D5_A2D_2
        en, du: D5A2D2 = ~ArmDel80 && ElevLow70 && ~PartIn70;
      state D5_SuctOff
        entry: D5A2D2=false; D5SuctOn=false;
        en, du: D5SuctOff = PartStuck80;
      state D5_PartDel
        entry: D5SuctOff=false; D5Transport=false; D5PartStuckM=false; D5PartDelEdge=true;
      state D5_N3_T3
        entry: D5PartDelEdge=false;
      state D5_N3_A2M_2
        en, du: D5A2M2 = ~ArmMag80;
      state D5_N4_Reset
        entry: D5A2M2=false; D5On=false;
      (default) -> OB1_N8_Off
      OB1_N8_Off -> DIST_Ctrl.FB5_Continuous.FB5_Wait : [DistInit85 && SimControl_80.SC_85_Continuous]
      D5_N4_Reset -> DIST_Ctrl.FB5_Continuous.FB5_Wait
      DIST_Ctrl.FB5_Continuous.FB5_Wait -> FB5_N1_AutoOn : [(SimSensors_80.SS_81_Start || SimControl_80.SC_85_Start || (CRouteIn80 && KeyPos81)) && ElevLow70 && ~PartIn70 && PartinMag80]
      FB5_N1_AutoOn -> D5_A2D_1
      D5_A2D_1 -> D5_PistFwd : [ArmDel80 && PistBck80]
      D5_PartDel -> D5_PistFwd [order 1] : [~MagEmpty80 && PistBck80 && ArmDel80]{D5PartDelEdge=false; D5PistFwd=true;}
      D5_PistFwd -> D5_Transport : [PistFwd80]
      D5_Transport -> D5_A2M_1
      D5_A2M_1 -> D5_SuctOn : [ArmMag80]
      D5_SuctOn -> D5_PartStuck : [PartStuck80]
      D5_PartStuck -> D5_A2D_2
      D5_A2D_2 -> D5_SuctOff : [ArmDel80]
      D5_SuctOff -> D5_PartDel : [~PartStuck80]
      D5_PartDel -> D5_N3_T3 [order 2] : [MagEmpty80 && PistBck80 && ArmDel80]
      D5_N3_T3 -> D5_N3_A2M_2 : after(T_DIST_T3,sec)
      D5_N3_A2M_2 -> D5_N4_Reset : [ArmMag80]
    state FB6_Counted [parallel]
      settings: executionOrder=6
      state OB1_N9_Off
      state FB6_Wait
      state FB6_N1_N2_LoadC2
        entry: cnt87 = RQ_PARTS + 1; D6On = cnt87 > 0;
      state D6_A2D_1
        en, du: D6A2D1 = ~ArmDel80 && ElevLow70 && ~PartIn70;
      state D6_PistFwd
        entry: D6A2D1=false; D6PistFwd=true;
      state D6_Transport
        entry: D6Transport=true; D6PistFwd=false;
      state D6_A2M_1
        en, du: D6A2M1 = ~ArmMag80;
      state D6_SuctOn
        entry: D6A2M1=false; D6SuctOn=true;
      state D6_PartStuck
        entry: D6PartStuckM=true;
      state D6_A2D_2
        en, du: D6A2D2 = ~ArmDel80 && ElevLow70 && ~PartIn70;
      state D6_SuctOff
        entry: D6A2D2=false; D6SuctOn=false;
        en, du: D6SuctOff = PartStuck80;
      state D6_PartDel
        entry: D6SuctOff=false; D6PartDel=true; D6Transport=false; D6PartStuckM=false;
      state D6_A2M_2
        en, du: D6A2M2 = ~ArmMag80;
      state D6_N4_Wait
        entry: D6A2M2=false;
      state D6_N4_DecCount
        entry: cnt87 = max(cnt87 - 1, 0); D6On = cnt87 > 0;
      state D6_N5_NewCycle
        entry: D6PartDel=false;
      (default) -> OB1_N9_Off
      OB1_N9_Off -> DIST_Ctrl.FB6_Counted.FB6_Wait : [DistInit85 && SimControl_80.SC_85_Counted]
      D6_N5_NewCycle -> DIST_Ctrl.FB6_Counted.FB6_Wait [order 2] : [~D6On]
      DIST_Ctrl.FB6_Counted.FB6_Wait -> FB6_N1_N2_LoadC2 : [(SimSensors_80.SS_81_Start || SimControl_80.SC_85_Start || (CRouteIn80 && KeyPos81)) && ArmMag80 && ElevLow70 && ~PartIn70 && PartinMag80 && cnt80 >= RQ_PARTS]
      FB6_N1_N2_LoadC2 -> D6_A2D_1
      D6_N5_NewCycle -> D6_A2D_1 [order 1] : [D6On]
      D6_A2D_1 -> D6_PistFwd : [ArmDel80 && PistBck80]
      D6_PistFwd -> D6_Transport : [PistFwd80]
      D6_Transport -> D6_A2M_1
      D6_A2M_1 -> D6_SuctOn : [ArmMag80]
      D6_SuctOn -> D6_PartStuck : [PartStuck80]
      D6_PartStuck -> D6_A2D_2
      D6_A2D_2 -> D6_SuctOff : [ArmDel80]
      D6_SuctOff -> D6_PartDel : [~PartStuck80]
      D6_PartDel -> D6_A2M_2
      D6_A2M_2 -> D6_N4_Wait : [ArmMag80]
      D6_N4_Wait -> D6_N4_DecCount [order 1] : [(D6PartDel && TEST_MODE == 1) || (RQPartDel70 && TEST_MODE == 2)]
      D6_N4_Wait -> D6_N5_NewCycle [order 2] : [RQWrong70 && TEST_MODE == 2]
      D6_N4_DecCount -> D6_N5_NewCycle : after(T_DIST_T3,sec)
    state OB1_N10_N11 [parallel]
      settings: executionOrder=3
      state OB1_N10_Wait
      state OB1_N11_PartDel
        entry: PartDel85=true; SimControl_80.SC_85_Part_Del=true; nDistDel = nDistDel + 1;
      state OB1_N10_Hold
        entry: PartDel85=false; SimControl_80.SC_85_Part_Del=false;
      (default) -> OB1_N10_Wait
      OB1_N10_Hold -> OB1_N10_Wait : [~D4PartDel && ~D5PartDelEdge && ~D6PartDel]
      OB1_N10_Wait -> OB1_N11_PartDel : [D4PartDel || D5PartDelEdge || D6PartDel]
      OB1_N11_PartDel -> OB1_N10_Hold : after(T_DIST_T4,sec)
    state FB3_Map80 [parallel]
      settings: executionOrder=7
      state FB3_Map
        during: PistAdv80 = KeyPos81 && (D4PistFwd || D5PistFwd || D6PistFwd);
        SuctOn80 = KeyPos81 && (D4SuctOn || D5SuctOn || D6SuctOn);
        SuctOff80 = KeyPos81 && (D4SuctOff || D5SuctOff || D6SuctOff);
        A2D80 = KeyPos81 && (D4A2D1 || D4A2D2 || D5A2D1 || D5A2D2 || D6A2D1 || D6A2D2);
        A2M80 = KeyPos81 && (FB1A2M2_80 || D4A2M1 || D4A2M2 || D5A2M1 || D5A2M2 || D6A2M1 || D6A2M2);
        SimActuators_80.SA_80_Pist_Adv = PistAdv80; SimActuators_80.SA_80_Suction_On = SuctOn80; SimActuators_80.SA_80_Suction_Off = SuctOff80;
        SimActuators_80.SA_80_Arm_2_Del = A2D80; SimActuators_80.SA_80_Arm_2_Mag = A2M80;
        SimActuators_80.SA_81_Led_Start = KeyPos81 && DistInit85; SimActuators_80.SA_81_Led_Extra1 = PartDel85;
      (default) -> DIST_Ctrl.FB3_Map80.FB3_Map
  state DIST_Plant [parallel]
    entry: KeyPos81=true; magCount = MAG_PARTS0; ArmMag80=true; PistBck80=true;
    MagFull80 = magCount >= MAG_CAP; MagEmpty80 = magCount <= 0;
    SimSensors_80.SS_81_Key_Pos=true; SimSensors_80.SS_81_Start=false; SimSensors_80.SS_81_Stop=false; SimSensors_80.SS_81_Reset=false;
    SimSensors_80.SS_81_Panel_I4=false; SimSensors_80.SS_81_Panel_I5=false; SimSensors_80.SS_81_Panel_I6=false; SimSensors_80.SS_81_Panel_I7=false;
    settings: executionOrder=10
    state Arm [parallel]
      settings: executionOrder=1
      state Arm_AtMag
        entry: ArmMag80=true; ArmDel80=false;
      state Arm_ToDel
        entry: tArm = 0; ArmLoaded = PartInArm;
        during: tArm = tArm + Ts_SIM;
        if ArmLoaded, ArmMag80 = tArm < t_d_magoff_load; else, ArmMag80 = tArm < t_d_magoff_empty; end
      state Arm_AtDel
        entry: ArmDel80=true; ArmMag80=false; SStation70=true;
      state Arm_ToMag
        entry: tArm = 0;
        during: tArm = tArm + Ts_SIM; ArmDel80 = tArm < t_d_deloff;
        if tArm >= t_d_sst_off, SStation70 = false; end
      (default) -> Arm_AtMag
      Arm_ToMag -> Arm_AtMag [order 1] : [tArm >= t_d_a2m]
      Arm_AtMag -> Arm_ToDel : [A2D80 && ~A2M80]
      Arm_ToMag -> Arm_ToDel [order 2] : [A2D80 && ~A2M80]
      Arm_ToDel -> Arm_AtDel [order 1] : [(~ArmLoaded && tArm >= t_d_a2d_empty) || (ArmLoaded && tArm >= t_d_a2d_load)]
      Arm_ToDel -> Arm_ToMag [order 2] : [A2M80 && ~A2D80]
      Arm_AtDel -> Arm_ToMag : [A2M80 && ~A2D80]
    state Suction [parallel]
      settings: executionOrder=3
      state Suct_Idle
      state Suct_Gripping
      state Suct_Holding
        entry: PartStuck80=true; PartInArm=true; PartAtPickup=false;
      state Suct_Release
      state Suct_Dropped
        entry: PartStuck80=false; PartInArm=false;
        if ArmDel80, PartIn70 = true; testColor = PART_COLORS(min(nTestIn + 1, numel(PART_COLORS))); nTestIn = nTestIn + 1; SInd70 = (testColor == 3); end
      (default) -> Suct_Idle
      Suct_Dropped -> Suct_Idle
      Suct_Idle -> Suct_Gripping : [SuctOn80 && ArmMag80 && PartAtPickup]
      Suct_Gripping -> Suct_Holding : after(t_d_suct,sec)
      Suct_Holding -> Suct_Release : [~SuctOn80]
      Suct_Release -> Suct_Dropped : after(t_d_release,sec)
    state MagPiston [parallel]
      settings: executionOrder=2
      state DPist_Back
        entry: PistBck80=true; PistFwd80=false;
      state DPist_Fwd
        entry: tPistD = 0;
        during: tPistD = tPistD + Ts_SIM; PistBck80 = tPistD < t_d_pist_bckoff;
        if tPistD >= t_d_pist_fwd && ~PistFwd80
        PistFwd80 = true;
        if magCount > 0, magCount = magCount - 1; PartAtPickup = true; end
        end
      state DPist_Return
        entry: PistFwd80=false;
      (default) -> DPist_Back
      DPist_Return -> DPist_Back : after(t_d_pist_back,sec)
      DPist_Back -> DPist_Fwd : [PistAdv80]
      DPist_Fwd -> DPist_Return : [~PistAdv80]
    state Sensors_Out80 [parallel]
      settings: executionOrder=4
      state S80_Map
        en, du: MagFull80 = magCount >= MAG_CAP; MagEmpty80 = magCount <= 0;
        SimSensors_80.SS_80_Arm_Mag = ArmMag80; SimSensors_80.SS_80_Arm_Del = ArmDel80; SimSensors_80.SS_80_Pist_Bck = PistBck80;
        SimSensors_80.SS_80_Pist_Fwd = PistFwd80; SimSensors_80.SS_80_Part_Stuck = PartStuck80;
        SimSensors_80.SS_80_Mag_Full = MagFull80; SimSensors_80.SS_80_Mag_Empty = MagEmpty80;
      (default) -> S80_Map
  state PROC_Ctrl [parallel]
    entry: SimControl_100.SC_102_Profibus=false; SimControl_100.SC_103_RQ_Turns = RQ_TURNS; SimControl_100.SC_105_Initialization=false; SimControl_100.SC_105_Start=false;
    SimControl_100.SC_105_Part_ready=false; SimControl_100.SC_105_Test_Ok=false; SimControl_100.SC_105_Test_Fail=false; SimControl_100.SC_106_RT_Counter=0;
    SimControl_100.SC_105_Test = (PROC_MODE == 1); SimControl_100.SC_105_TestDrill = (PROC_MODE == 2); SimControl_100.SC_105_Rotation = (PROC_MODE == 3);
    SimActuators_100.SA_100_Drill_On=false; SimActuators_100.SA_100_RT_On=false; SimActuators_100.SA_100_Drill_Down=false; SimActuators_100.SA_100_Drill_Up=false; SimActuators_100.SA_100_Drill_Pin=false; SimActuators_100.SA_100_Test_Pin=false; SimActuators_100.SA_101_Led_Start=false; SimActuators_100.SA_101_Led_Reset=false; SimActuators_100.SA_101_Led_Extra1=false; SimActuators_100.SA_101_Led_Extra2=false; SimActuators_100.SA_101_Panel_O4=false; SimActuators_100.SA_101_Panel_O5=false; SimActuators_100.SA_101_Panel_O6=false; SimActuators_100.SA_101_Panel_O7=false;
    settings: executionOrder=11
    state FB1_Init100 [parallel]
      settings: executionOrder=1
      state FB1_N2_DrillUp
        entry: SimControl_100.SC_102_Profibus=true; ProcInit=false;
        en, du: P1DrillUp = ~SDrillHigh100;
      state FB1_N3_Empty1
        entry: P1DrillUp=false; P1DrillH=true;
      state FB1_N4_Rotate3
        entry: P1Empty1=true; cntRT = 3; P1RT1=true;
      state FB1_N5_Empty2
        entry: P1RT1=false;
      state FB1_N12_InitOk
        entry: P1Empty2=true; ProcInit=true; SimControl_100.SC_105_Initialization=true;
      state FB1_N6_N11_Clear
        entry: ProcInit=false;
      (default) -> FB1_N2_DrillUp
      FB1_N2_DrillUp -> FB1_N3_Empty1 : [SDrillHigh100]
      FB1_N3_Empty1 -> FB1_N4_Rotate3 [order 1] : [~RtOn100 && RTSens100 && ~PInit100 && ~PDrill100 && ~PTest100]
      FB1_N3_Empty1 -> FB1_N6_N11_Clear [order 2] : [~RtOn100 && RTSens100 && (PInit100 || PDrill100 || PTest100)]
      FB1_N4_Rotate3 -> FB1_N5_Empty2 : [cntRT <= 0]
      FB1_N5_Empty2 -> FB1_N12_InitOk [order 1] : [~RtOn100 && RTSens100 && ~PInit100 && ~PDrill100 && ~PTest100]
      FB1_N5_Empty2 -> FB1_N6_N11_Clear [order 2] : [~RtOn100 && RTSens100 && (PInit100 || PDrill100 || PTest100)]
    state OB1_N4_N8 [parallel]
      settings: executionOrder=2
      state OB1_N4_N8_Map
        en, du: PartReady100 = P4Ready || P5Ready || P6Ready; SimControl_100.SC_105_Part_ready = PartReady100;
        if RtOn100 && RTSens100 && ~prevRTSens100, cnt106 = cnt106 + 1; end
        if ~RtOn100, cnt106 = 0; end
        if RTSens100 && ~prevRTSens100 && cntRT > 0, cntRT = cntRT - 1; end
        prevRTSens100 = RTSens100; SimControl_100.SC_106_RT_Counter = cnt106;
      (default) -> OB1_N4_N8_Map
    state FB4_Test [parallel]
      settings: executionOrder=3
      state OB1_N5_Off
      state FB4_Wait
      state FB4_N1_StartTest
        entry: P4Start=true; SimControl_100.SC_105_Test_Ok=false; SimControl_100.SC_105_Test_Fail=false; P4OK=false; P4Fail=false;
      state FB4_N2_SpinToTest
        entry: cntRT = 4; P4RT=true;
      state FB4_N3_T4_TestDelay
        entry: P4RT=false;
      state FB4_N4_TestPin
        entry: P4Pin=true;
      state FB4_N5_N6_Result
        entry: P4OK = PTestOk100; P4Fail = ~PTestOk100;
        SimControl_100.SC_105_Test_Ok = P4OK; SimControl_100.SC_105_Test_Fail = P4Fail;
      state FB4_N7_SpinToCollect
        entry: P4Pin=false; cntRT = 2; P4RT=true;
      state FB4_N8_PartReady
        entry: P4RT=false; P4Ready=true;
      state FB4_N9_PickedUp
        entry: P4Ready=false; P4OK=false; P4Fail=false; P4Start=false;
      (default) -> PROC_Ctrl.FB4_Test.OB1_N5_Off
      PROC_Ctrl.FB4_Test.OB1_N5_Off -> PROC_Ctrl.FB4_Test.FB4_Wait : [ProcInit && SimControl_100.SC_105_Test]
      FB4_N9_PickedUp -> PROC_Ctrl.FB4_Test.FB4_Wait
      PROC_Ctrl.FB4_Test.FB4_Wait -> FB4_N1_StartTest : [PInit100 && ClawHigh90 && RTSens100 && ~RtOn100]
      FB4_N1_StartTest -> FB4_N2_SpinToTest
      FB4_N2_SpinToTest -> FB4_N3_T4_TestDelay : [cntRT <= 0]
      FB4_N3_T4_TestDelay -> FB4_N4_TestPin : [~RtOn100 && PTest100 && RTSens100]
      FB4_N4_TestPin -> FB4_N5_N6_Result : after(T_PROC_T5,sec)
      FB4_N5_N6_Result -> FB4_N7_SpinToCollect
      FB4_N7_SpinToCollect -> FB4_N8_PartReady : [cntRT <= 0]
      FB4_N8_PartReady -> FB4_N9_PickedUp : [ClawDel90 && ClawLow90 && PartInClaw90]
    state FB5_TestDrill [parallel]
      settings: executionOrder=4
      state OB1_N6_Off
      state FB5_Wait
      state FB5_N1_StartTD
        entry: P5Start=true; SimControl_100.SC_105_Test_Ok=false; SimControl_100.SC_105_Test_Fail=false; P5OK=false; P5Fail=false; P5DrillOk=false;
      state FB5_N2_SpinToTest
        entry: cntRT = 4; P5RT=true;
      state FB5_N3_T4_TestDelay
        entry: P5RT=false;
      state FB5_N4_TestPin
        entry: P5Pin=true;
      state FB5_N5_N6_Result
        entry: P5OK = PTestOk100; P5Fail = ~PTestOk100;
        SimControl_100.SC_105_Test_Ok = P5OK; SimControl_100.SC_105_Test_Fail = P5Fail;
      state FB5_N7_SpinToDrill
        entry: P5Pin=false; cntRT = 1; P5RT=true;
      state FB5_N8_PinLowerDrill
        entry: P5RT=false; P5DrillPin=true; P5LDrill=true;
      state FB5_N9_N10_T8_Drill
        entry: P5TDrill=true;
      state FB5_N11_RaiseDrill
        entry: P5TDrill=false; P5LDrill=false; P5RDrill=true;
      state FB5_N12_N13_SpinFinal
        entry: P5DrillPin=false; P5RDrill=false; P5DrillOk=true; cntRT = 1; P5RT=true;
      state FB5_N14_SpinFinalFail
        entry: P5Pin=false; cntRT = 2; P5RT=true;
      state FB5_N15_PartReady
        entry: P5RT=false; P5Ready=true;
      state FB5_N16_PickedUp
        entry: P5Ready=false; P5OK=false; P5Fail=false; P5DrillOk=false; P5Start=false;
      (default) -> OB1_N6_Off
      OB1_N6_Off -> PROC_Ctrl.FB5_TestDrill.FB5_Wait : [ProcInit && SimControl_100.SC_105_TestDrill]
      FB5_N16_PickedUp -> PROC_Ctrl.FB5_TestDrill.FB5_Wait
      PROC_Ctrl.FB5_TestDrill.FB5_Wait -> FB5_N1_StartTD : [PInit100 && ClawHigh90 && RTSens100 && ~RtOn100]
      FB5_N1_StartTD -> FB5_N2_SpinToTest
      FB5_N2_SpinToTest -> FB5_N3_T4_TestDelay : [cntRT <= 0]
      FB5_N3_T4_TestDelay -> FB5_N4_TestPin : [~RtOn100 && PTest100 && RTSens100]
      FB5_N4_TestPin -> FB5_N5_N6_Result : after(T_PROC_T5,sec)
      FB5_N5_N6_Result -> FB5_N7_SpinToDrill [order 1] : [P5OK]
      FB5_N5_N6_Result -> FB5_N14_SpinFinalFail [order 2] : [P5Fail]
      FB5_N7_SpinToDrill -> FB5_N8_PinLowerDrill : [cntRT <= 0]
      FB5_N8_PinLowerDrill -> FB5_N9_N10_T8_Drill : [SDrillLow100]
      FB5_N9_N10_T8_Drill -> FB5_N11_RaiseDrill : after(T_PROC_T8,sec)
      FB5_N11_RaiseDrill -> FB5_N12_N13_SpinFinal : [SDrillHigh100]
      FB5_N12_N13_SpinFinal -> FB5_N15_PartReady : [cntRT <= 0]
      FB5_N14_SpinFinalFail -> FB5_N15_PartReady : [cntRT <= 0]
      FB5_N15_PartReady -> FB5_N16_PickedUp : [ClawDel90 && ClawLow90 && PartInClaw90]
    state FB6_Rotation [parallel]
      settings: executionOrder=5
      state OB1_N7_Off
      state FB6_Wait
      state FB6_N1_StartR
        entry: P6Start=true; P6RotOK=false;
      state FB6_N2_Spin6
        entry: cntRT = 6; P6RT=true;
      state FB6_N3_N4_RotationOK
        entry: P6RT=false; P6RotOK=true; P6Ready=true;
      state FB6_N5_PickedUp
        entry: P6Ready=false; P6RotOK=false; P6Start=false;
      (default) -> PROC_Ctrl.FB6_Rotation.OB1_N7_Off
      PROC_Ctrl.FB6_Rotation.OB1_N7_Off -> PROC_Ctrl.FB6_Rotation.FB6_Wait : [ProcInit && SimControl_100.SC_105_Rotation]
      FB6_N5_PickedUp -> PROC_Ctrl.FB6_Rotation.FB6_Wait
      PROC_Ctrl.FB6_Rotation.FB6_Wait -> FB6_N1_StartR : [PInit100 && ClawHigh90 && ~RtOn100]
      FB6_N1_StartR -> FB6_N2_Spin6
      FB6_N2_Spin6 -> FB6_N3_N4_RotationOK : [cntRT <= 0]
      FB6_N3_N4_RotationOK -> FB6_N5_PickedUp : [ClawDel90 && ClawLow90 && PartInClaw90]
    state FB3_Map100 [parallel]
      settings: executionOrder=6
      state FB3_Map
        during: RtOn100 = KeyPos101 && ((P1RT1 && cntRT > 0 && (ClawHigh90 || ~ClawDel90)) || (P4RT && cntRT > 0) || (P5RT && cntRT > 0) || (P6RT && cntRT > 0));
        DrillDown100 = KeyPos101 && P5LDrill; DrillUp100 = KeyPos101 && (P1DrillUp || P5RDrill);
        DrillPin100 = KeyPos101 && P5DrillPin; DrillOn100 = KeyPos101 && P5TDrill; TestPin100 = KeyPos101 && (P4Pin || P5Pin);
        SimActuators_100.SA_100_RT_On = RtOn100; SimActuators_100.SA_100_Drill_Down = DrillDown100; SimActuators_100.SA_100_Drill_Up = DrillUp100;
        SimActuators_100.SA_100_Drill_Pin = DrillPin100; SimActuators_100.SA_100_Drill_On = DrillOn100; SimActuators_100.SA_100_Test_Pin = TestPin100;
        SimActuators_100.SA_101_Led_Start = KeyPos101 && ProcInit; SimActuators_100.SA_101_Led_Extra1 = PartReady100;
      (default) -> PROC_Ctrl.FB3_Map100.FB3_Map
  state PROC_Plant [parallel]
    entry: KeyPos101=true; RTSens100=true; SDrillHigh100=true;
    SimSensors_100.SS_101_Key_Pos=true; SimSensors_100.SS_101_Start=false; SimSensors_100.SS_101_Stop=false; SimSensors_100.SS_101_Reset=false;
    SimSensors_100.SS_101_Panel_I4=false; SimSensors_100.SS_101_Panel_I5=false; SimSensors_100.SS_101_Panel_I6=false; SimSensors_100.SS_101_Panel_I7=false;
    settings: executionOrder=12
    state Table [parallel]
      settings: executionOrder=1
      state RT_Stopped
      state RT_Moving
        entry: tRt = 0;
        during: tRt = tRt + Ts_SIM;
        if tRt >= t_rt_step, tRt = 0; RTSens100 = true; partOff = mod(partOff + 1, 6);
        elseif tRt >= t_rt_hi, RTSens100 = false; end
      (default) -> RT_Stopped
      RT_Moving -> RT_Stopped : [~RtOn100]
      RT_Stopped -> RT_Moving : [RtOn100]
    state Probe_Sensors [parallel]
      settings: executionOrder=3
      state Sens_Map
        en, du: PInit100 = PartOnTable && partOff == 0 && ~RtOn100;
        PTest100 = PartOnTable && partOff == 4 && ~RtOn100; PDrill100 = PartOnTable && partOff == 5 && ~RtOn100;
        SimSensors_100.SS_100_PInit_Pos = PInit100; SimSensors_100.SS_100_PTest_Pos = PTest100; SimSensors_100.SS_100_PDrill_Pos = PDrill100;
        SimSensors_100.SS_100_RT_Sensor = RTSens100; SimSensors_100.SS_100_SDrill_High = SDrillHigh100; SimSensors_100.SS_100_SDrill_Low = SDrillLow100;
        SimSensors_100.SS_100_PTest_Ok = PTestOk100;
      (default) -> Sens_Map
    state Drill [parallel]
      settings: executionOrder=2
      state Drill_Up
        entry: SDrillHigh100=true; SDrillLow100=false;
      state Drill_GoingDown
        entry: SDrillHigh100=false;
      state Drill_Low
        entry: SDrillLow100=true;
      state Drill_GoingUp
        entry: SDrillLow100=false;
      (default) -> Drill_Up
      Drill_GoingUp -> Drill_Up : after(t_drill_up,sec)
      Drill_Up -> Drill_GoingDown : [DrillDown100 && ~DrillUp100]
      Drill_GoingDown -> Drill_Low : after(t_drill_down,sec)
      Drill_Low -> Drill_GoingUp : [DrillUp100]
    state TestProbe [parallel]
      settings: executionOrder=4
      state Probe_Up
        entry: PTestOk100=false;
      state Probe_Down
      state Probe_Read
        entry: PTestOk100 = PTest100 && PROC_TEST_OK(min(max(procIdx,1), numel(PROC_TEST_OK))) == 1;
      (default) -> Probe_Up
      Probe_Read -> Probe_Up : [~TestPin100]
      Probe_Up -> Probe_Down : [TestPin100]
      Probe_Down -> Probe_Read : after(t_ptest_ok,sec)
  state HD2_Feed_PROVISORIO [parallel]
    settings: executionOrder=13
    state H2P_Idle
      entry: ClawHigh90=true; ClawLow90=false; ClawDel90=false; PartInClaw90=false;
    state H2P_AtDel
      entry: ClawDel90=true; PartInClaw90=true;
    state H2P_Down
      entry: ClawHigh90=false;
    state H2P_LowPlace
      entry: ClawLow90=true; PartOnTable=true; partOff=0; nProcIn = nProcIn + 1; procIdx = nProcIn;
    state H2P_Up
      entry: ClawLow90=false; PartInClaw90=false;
    state H2P_HighWait
      entry: ClawHigh90=true;
    state H2P_PickDown
      entry: ClawHigh90=false;
    state H2P_PickLow
      entry: ClawLow90=true; PartInClaw90=true; PartOnTable=false;
    state H2P_PickUp
      entry: ClawLow90=false;
    state H2P_PickHigh
      entry: ClawHigh90=true;
    state H2P_Leave
      entry: ClawDel90=false; nProcOut = nProcOut + 1;
    (default) -> H2P_Idle
    H2P_Leave -> H2P_Idle : after(t_h2_return,sec)
    H2P_Idle -> H2P_AtDel : [ProcInit && nProcIn < N_PARTS]
    H2P_AtDel -> H2P_Down : after(t_h2_down,sec)
    H2P_Down -> H2P_LowPlace : after(t_h2_low,sec)
    H2P_LowPlace -> H2P_Up : after(t_h2_up,sec)
    H2P_Up -> H2P_HighWait : after(t_h2_high,sec)
    H2P_HighWait -> H2P_PickDown : [PartReady100]
    H2P_PickDown -> H2P_PickLow : after(t_h2_pick_down,sec)
    H2P_PickLow -> H2P_PickUp : after(t_h2_pick_low,sec)
    H2P_PickUp -> H2P_PickHigh : after(t_h2_pick_up,sec)
    H2P_PickHigh -> H2P_Leave : after(t_h2_leave,sec)
  data: SimActuators_20 output Bus: B_SimActuators_20; SimControl_20 output Bus: B_SimControl_20; SimSensors_20 output Bus: B_SimSensors_20; SimActuators_50 output Bus: B_SimActuators_50; SimASi_50 output Bus: B_SimASi_50; SimControl_50 output Bus: B_SimControl_50; SimSensors_50 output Bus: B_SimSensors_50; SimActuators_60 output Bus: B_SimActuators_60; SimControl_60 output Bus: B_SimControl_60; SimSensors_60 output Bus: B_SimSensors_60; Ts_SIM parameter double; T_HD1_T1 parameter double; T_CONV_T6 parameter double; t_v_down parameter double; t_v_up parameter double; t_h_del parameter double; t_h_cart parameter double; t_grip parameter double; t_conv parameter double; t_leave parameter double; N_PARTS parameter double; SORT_MODE parameter double; T_SORT_ID parameter double; T_SORT_T7 parameter double; t_s_spart_off parameter double; t_s_photo parameter double; t_s_ind parameter double; t_s_ind_off parameter double; t_s_photo_off parameter double; t_s_pass1 parameter double; t_s_pass2 parameter double; t_s_pass3 parameter double; t_s_pp parameter double; t_sl1_fwd parameter double; t_sl1_bck parameter double; t_sl2_fwd parameter double; t_sl2_bck parameter double; PART_COLORS parameter double; SORT_MAP parameter double; PartOnCart local boolean =false; CartAt29 local boolean =false; CRouteIn54 local boolean =false; Claw2CartCmd local boolean =false; FB1Init local boolean =false; FB1Conv local boolean =false; FB1IDPin local boolean =false; FBSel local boolean =false; ConvOn60 local boolean =false; TrigConv local boolean =false; Lever1 local boolean =false; Lever2 local boolean =false; PassStr local boolean =false; PinSort local boolean =false; PartDel local boolean =false; nCart local double =0; nDone local double =0; nSortIn local double =0; sortColor local double =0; sortExit local double =0; cID local double =0; xSort local double =0; SimActuators_70 output Bus: B_SimActuators_70; SimASi_70 output Bus: B_SimASi_70; SimControl_70 output Bus: B_SimControl_70; SimSensors_70 output Bus: B_SimSensors_70; TEST_MODE parameter double; T_TEST_T1 parameter double; T_TEST_T2 parameter double; T_TEST_T8 parameter double; T_TEST_T3 parameter double; T_TEST_T5 parameter double; T_TEST_T6 parameter double; T_TEST_T7 parameter double; T_CONV24_T1 parameter double; t_t_up parameter double; t_t_up_lowoff parameter double; t_t_up_ind parameter double; t_t_up_sst parameter double; t_t_metal_off parameter double; t_t_height_pre parameter double; t_t_down parameter double; t_t_down_highoff parameter double; t_t_down_sst parameter double; t_t_down_ind parameter double; t_t_ej_spart parameter double; t_t_pist_fwd parameter double; t_t_pist_back parameter double; t_t_ej_cart parameter double; t_24_arrive parameter double; t_24_count parameter double; t_24_req parameter double; t_24_croute_in0 parameter double; t_24_croute_in parameter double; t_24_pist_bck parameter double; t_24_optic_off parameter double; t_24_leave parameter double; RQ_DELIVERY parameter double; FB1Init70 local boolean =false; FB1ElevDown70 local boolean =false; FB1PistAdv70 local boolean =false; IdenDel local boolean =false; IdenProc local boolean =false; EjectProc local boolean =false; ReturnElev local boolean =false; FB4ElevUp local boolean =false; FB4ElevDown local boolean =false; FB4PistFwd local boolean =false; FB4Air local boolean =false; FB4CartFull local boolean =false; ReqDel local boolean =false; IdenColor local boolean =false; PartOk local boolean =false; EjectOk local boolean =false; PartDiff local boolean =false; EjectBad local boolean =false; FB5ElevUp local boolean =false; FB5ElevDown1 local boolean =false; FB5ElevDown2 local boolean =false; FB5PistFwd1 local boolean =false; FB5PistFwd2 local boolean =false; FB5Air local boolean =false; FB5CartFull local boolean =false; idA70 local boolean =false; idB70 local boolean =false; PartDel70 local boolean =false; RQPartDel70 local boolean =false; RQWrong70 local boolean =false; RQ1_70 local boolean =false; RQ2_70 local boolean =false; RouteOut74 local boolean =false; NoCart74 local boolean =false; CartFull74 local boolean =false; ElevUp70 local boolean =false; ElevDown70 local boolean =false; Eject70 local boolean =false; Air70 local boolean =false; CRouteIn80 local boolean =false; CRouteIn74 local boolean =false; CartStat24 local boolean =false; Optic24 local boolean =false; PistBck24 local boolean =false; ArmMag80 local boolean =false; KeyPos71 local boolean =false; PartToCart local boolean =false; CartHasPart local boolean =false; PartIn70 local boolean =false; ElevLow70 local boolean =false; ElevHigh70 local boolean =false; SInd70 local boolean =false; Height70 local boolean =false; PistBck70 local boolean =false; SStation70 local boolean =false; nTest local double =0; nTestIn local double =0; nReject local double =0; testColor local double =0; tElev local double =0; tPist local double =0; SimActuators_80 output Bus: B_SimActuators_80; SimControl_80 output Bus: B_SimControl_80; SimSensors_80 output Bus: B_SimSensors_80; DIST_MODE parameter double; RQ_PARTS parameter double; MAG_PARTS0 parameter double; MAG_CAP parameter double; T_DIST_T1 parameter double; T_DIST_T2 parameter double; T_DIST_T3 parameter double; T_DIST_T4 parameter double; t_d_a2d_empty parameter double; t_d_a2d_load parameter double; t_d_magoff_empty parameter double; t_d_magoff_load parameter double; t_d_a2m parameter double; t_d_deloff parameter double; t_d_sst_off parameter double; t_d_pist_fwd parameter double; t_d_pist_bckoff parameter double; t_d_pist_back parameter double; t_d_suct parameter double; t_d_release parameter double; DistInit85 local boolean =false; FB1MagEmpty80 local boolean =false; FB1MagFull80 local boolean =false; FB1A2M2_80 local boolean =false; PartinMag80 local boolean =false; PartDel85 local boolean =false; ArmDel80 local boolean =false; PistBck80 local boolean =false; PistFwd80 local boolean =false; PartStuck80 local boolean =false; MagFull80 local boolean =false; MagEmpty80 local boolean =false; KeyPos81 local boolean =false; A2D80 local boolean =false; A2M80 local boolean =false; PistAdv80 local boolean =false; SuctOn80 local boolean =false; SuctOff80 local boolean =false; PartAtPickup local boolean =false; PartInArm local boolean =false; ArmLoaded local boolean =false; prevMagFull80 local boolean =false; prevPistFwd80 local boolean =false; D4On local boolean =false; D4Transport local boolean =false; D4PartStuckM local boolean =false; D4PartDel local boolean =false; D4A2D1 local boolean =false; D4A2D2 local boolean =false; D4A2M1 local boolean =false; D4A2M2 local boolean =false; D4PistFwd local boolean =false; D4SuctOn local boolean =false; D4SuctOff local boolean =false; D5On local boolean =false; D5Transport local boolean =false; D5PartStuckM local boolean =false; D5PartDelEdge local boolean =false; D5A2D1 local boolean =false; D5A2D2 local boolean =false; D5A2M1 local boolean =false; D5A2M2 local boolean =false; D5PistFwd local boolean =false; D5SuctOn local boolean =false; D5SuctOff local boolean =false; D6On local boolean =false; D6Transport local boolean =false; D6PartStuckM local boolean =false; D6PartDel local boolean =false; D6A2D1 local boolean =false; D6A2D2 local boolean =false; D6A2M1 local boolean =false; D6A2M2 local boolean =false; D6PistFwd local boolean =false; D6SuctOn local boolean =false; D6SuctOff local boolean =false; cnt80 local double =0; cnt87 local double =0; magCount local double =0; tArm local double =0; tPistD local double =0; tMagFull local double =0; tMagEmpty local double =0; nDistDel local double =0; SimActuators_100 output Bus: B_SimActuators_100; SimControl_100 output Bus: B_SimControl_100; SimSensors_100 output Bus: B_SimSensors_100; PROC_MODE parameter double; RQ_TURNS parameter double; T_PROC_T4 parameter double; T_PROC_T5 parameter double; T_PROC_T8 parameter double; t_rt_step parameter double; t_rt_hi parameter double; t_ptest_ok parameter double; t_drill_down parameter double; t_drill_up parameter double; t_h2_down parameter double; t_h2_low parameter double; t_h2_up parameter double; t_h2_high parameter double; t_h2_pick_down parameter double; t_h2_pick_low parameter double; t_h2_pick_up parameter double; t_h2_leave parameter double; t_h2_return parameter double; PROC_TEST_OK parameter double; ProcInit local boolean =false; P1DrillUp local boolean =false; P1DrillH local boolean =false; P1Empty1 local boolean =false; P1Empty2 local boolean =false; P1RT1 local boolean =false; PartReady100 local boolean =false; PartReadyM local boolean =false; P4Start local boolean =false; P4RT local boolean =false; P4Pin local boolean =false; P4OK local boolean =false; P4Fail local boolean =false; P4Ready local boolean =false; P5Start local boolean =false; P5RT local boolean =false; P5Pin local boolean =false; P5OK local boolean =false; P5Fail local boolean =false; P5DrillPin local boolean =false; P5LDrill local boolean =false; P5TDrill local boolean =false; P5RDrill local boolean =false; P5DrillOk local boolean =false; P5Ready local boolean =false; P6Start local boolean =false; P6RT local boolean =false; P6RotOK local boolean =false; P6Ready local boolean =false; RtOn100 local boolean =false; DrillDown100 local boolean =false; DrillUp100 local boolean =false; DrillPin100 local boolean =false; DrillOn100 local boolean =false; TestPin100 local boolean =false; KeyPos101 local boolean =false; RTSens100 local boolean =false; PInit100 local boolean =false; PTest100 local boolean =false; PDrill100 local boolean =false; SDrillHigh100 local boolean =false; SDrillLow100 local boolean =false; PTestOk100 local boolean =false; PartOnTable local boolean =false; prevRTSens100 local boolean =false; ClawHigh90 local boolean =false; ClawLow90 local boolean =false; ClawDel90 local boolean =false; PartInClaw90 local boolean =false; partOff local double =0; tRt local double =0; cntRT local double =0; cnt106 local double =0; nProcIn local double =0; nProcOut local double =0; procIdx local double =0
